simulink model "ADCSSimulator"  (R2024a)
settings: Solver=ode4  StartTime=0.0  StopTime=600  FixedStep=0.01  MaxStep=0.1  RelTol=1e-3  AbsTol=1e-3
values from neighbouring files (symbols this model uses):
  ActuatorAllocationMatrix = ActuatorPhysicalMatrix' * inv(ActuatorPhysicalMatrix * ActuatorPhysicalMatrix')    [set_Init.m]
  ActuatorPhysicalMatrix = [1, 0, 0, 0 ... (first row only)    [set_Init.m]
  albedo_irradiance = 300    [set_Init.m]
  b = 0    [set_Init.m]
  Cd = 2.2    [set_Init.m]
  h_bias = [0; 0; 0]    [set_Init.m]
  J = 4.0e-3 / 628    (= 6.36942675159e-06)    [set_Init.m]
  k_Bdot = ((4 * pi * 0.5236 * 0.0055) / (5677.2 * (4.5e-5)^2))    (= 3147.8423197)    [set_Init.m]
  K_E = K_T    (= 0.0022)    [set_Init.m]
  K_T = 0.0022    [set_Init.m]
  P0 = blkdiag(P0_att, P0_bias)    [set_Init.m]
  P0_att = eye(3) * initial_variance_rad2    [set_Init.m]
  PowerVoltageBus_01 = 3.3    [set_Init.m]
  PowerVoltageBus_02 = 3.3    [set_Init.m]
  PowerVoltageBus_03 = 3.3    [set_Init.m]
  PowerVoltageBus_04 = 3.3    [set_Init.m]
  PowerVoltageBus_05 = 3.3    [set_Init.m]
  PowerVoltageBus_06 = 3.3    [set_Init.m]
  PowerVoltageBus_07 = 3.3    [set_Init.m]
  PowerVoltageBus_08 = 3.3    [set_Init.m]
  PowerVoltageBus_09 = 3.3    [set_Init.m]
  PowerVoltageBus_10 = 3.3    [set_Init.m]
  PowerVoltageBus_11 = 3.3    [set_Init.m]
  PowerVoltageBus_12 = 0.0    (= 0)    [set_Init.m]
  PowerVoltageBus_13 = 0.0    (= 0)    [set_Init.m]
  PowerVoltageBus_14 = 0.0    (= 0)    [set_Init.m]
  PowerVoltageBus_15 = 0.0    (= 0)    [set_Init.m]
  R = 2.0    (= 2)    [set_Init.m]
  ressidual_m = [3e-4; -2e-4; 1e-4]    [set_Init.m]
  solar_irradiance = 1361    [set_Init.m]
  surface_areas = [A_xy, A_yz, A_xz, A_xy, A_yz, A_xz]    [set_Init.m]
  surface_normals_body = [eye(3) -eye(3)]    [set_Init.m]
  surface_positions_body = [       hx,   0,   0 ... (first row only)    [set_Init.m]
  surface_reflectivities = [0.9 0.8 0.9 0.9 0.9 0.9]    [set_Init.m]
  Switch_01 = 1    [set_Init.m]
  Switch_02 = 1    [set_Init.m]
  Switch_03 = 1    [set_Init.m]
  Switch_04 = 1    [set_Init.m]
  Switch_05 = 1    [set_Init.m]
  Switch_06 = 1    [set_Init.m]
  Switch_07 = 1    [set_Init.m]
  Switch_08 = 1    [set_Init.m]
  Switch_09 = 1    [set_Init.m]
  Switch_10 = 1    [set_Init.m]
  Switch_11 = 1    [set_Init.m]
  Switch_12 = 0    [set_Init.m]
  Switch_13 = 0    [set_Init.m]
  Switch_14 = 0    [set_Init.m]
  Switch_15 = 0    [set_Init.m]
  visSampleTime = 0.1    [set_Init.m]
undefined symbols (not defined in the file or in its folder): attitude, Controller, epoch, IAU, juliandate, Kd, km, Kp, m, rad, s, satellite, SGP4_parameters, simulator, UKF_parameters, WMM2020
libraries: sharedtransform x27, aerolibutil x22, aerolibconvert2 x18, simulink_extras x16, matrix_library x6, aerolibtransform2 x4, vrlib x2, aerolibgravity2 x2, aerolibobsolete x1, aerolibattitudesys x1, simulink x1
(part 5 of 8)

== system ADCSSimulator/ADCS/ADCS Hardware/Sensors/Gyroscope Model/Power Consumption Calculator ==
  note: $I_=\frac{V_{Bus}}{R} \\ P_{Consumption} =I V_{Bus}$
  Bus Voltage (V) : Inport
  Bus Creator : BusCreator  Inputs=2
  Gain1 : Gain  Gain=1/(satellite.Gyro.NominalVoltage^2/satellite.Gyro.NominalPower)
  Product : Product
  Gyro Power Consumption : Outport
  wires:
  Bus Voltage (V)/1 -> Gain1/1, Product/2
  Gain1/1 -> Product/1, Bus Creator/1  "Current (A)"
  Bus Creator/1 -> Gyro Power Consumption/1
  Product/1 -> Bus Creator/2  "Power Consumption (W)"

== system ADCSSimulator/ADCS/ADCS Hardware/Sensors/Sun Sensor Model/Init Data Wrapper ==
  Real Data : Inport
  Initial Value : Inport  Port=2
  Clock : Clock
  Switch : Switch  Threshold=1  SaturateOnIntegerOverflow=off  InputSameDT=off
  Wrapped Data : Outport
  wires:
  Clock/1 -> Switch/2
  Real Data/1 -> Switch/1
  Initial Value/1 -> Switch/3
  Switch/1 -> Wrapped Data/1

== system ADCSSimulator/ADCS/ADCS Hardware/Sensors/Sun Sensor Model/Normalizer8 ==
  A : Inport
  Divide : Product  Inputs=*/
  Dot Product : DotProduct  OutDataTypeStr=Inherit: Inherit via internal rule
  Sqrt1 : Sqrt
  Normalized(A) : Outport
  wires:
  Dot Product/1 -> Sqrt1/1
  A/1 -> Dot Product/2, Dot Product/1, Divide/1
  Sqrt1/1 -> Divide/2
  Divide/1 -> Normalized(A)/1

== system ADCSSimulator/ADCS/ADCS Hardware/Sensors/Sun Sensor Model/Power Consumption Calculator ==
  note: $I_=\frac{V_{Bus}}{R} \\ P_{Consumption} =I V_{Bus}$
  Bus Voltage (V) : Inport
  Bus Creator : BusCreator  Inputs=2
  Gain2 : Gain  Gain=1/(satellite.SS.NominalVoltage^2/satellite.SS.NominalPower)
  Product : Product
  SS Power Consumption : Outport
  wires:
  Bus Voltage (V)/1 -> Gain2/1, Product/2
  Gain2/1 -> Product/1, Bus Creator/1  "Current (A)"
  Bus Creator/1 -> SS Power Consumption/1
  Product/1 -> Bus Creator/2  "Power Consumption (W)"

== system ADCSSimulator/ADCS/ADCS Software/Attitude Control/Chart/Detumbling/Detumbling Algorithm ==
  Measured Magnetic Field [Body](T) : Inport
  Measured Angular Velocity [Body](rad/s) : Inport  Port=2
  Constant11 : Constant  Value=k_Bdot
  Cross Product : matrix_library/Cross Product
  Divide : Product  Inputs=*/
  Divide1 : Product  Inputs=*/
  Product : Product
  sqrt : Subsystem
  Detumbling: Magnetic Dipole Command : Outport
  wires:
  sqrt/1(sqrt(u)) -> Divide1/2, Divide/2  "||B||"
  Divide1/1 -> Detumbling: Magnetic Dipole Command/1  "k/||B||*omega*b"
  Product/1 -> Divide1/1  "k(omega*b)"
  Cross Product/1 -> Product/2  "omega*b"
  Divide/1 -> Cross Product/2  "b"
  Measured Angular Velocity [Body](rad/s)/1 -> Cross Product/1
  Constant11/1 -> Product/1
  Measured Magnetic Field [Body](T)/1 -> sqrt/1(u), Divide/1

== system ADCSSimulator/ADCS/ADCS Software/Attitude Control/Chart/Nadir_Pointing/Actuator Allocation & Feed-Forward ==
  m_cmd_raw_Am2 : Inport
  tau_req_Nm : Inport  Port=2
  B_meas_Body_T : Inport  Port=3
  Cross Product : matrix_library/Cross Product
  Saturation : Saturate  UpperLimit=satellite.MTQ.DPMoment  LowerLimit=-satellite.MTQ.DPMoment
  Sum : Sum  Inputs=|-+
  m_cmd_final : Outport
  tau_rw_cmd : Outport  Port=2
  wires:
  tau_req_Nm/1 -> Sum/2
  m_cmd_raw_Am2/1 -> Saturation/1
  Saturation/1 -> Cross Product/1, m_cmd_final/1
  B_meas_Body_T/1 -> Cross Product/2
  Cross Product/1 -> Sum/1
  Sum/1 -> tau_rw_cmd/1  "tau_net"

== system ADCSSimulator/ADCS/ADCS Software/Attitude Control/Chart/Nadir_Pointing/Momentum Management ==
  h_rw_Nms : Inport
  B_meas_Body_T : Inport  Port=2
  Cross Product : matrix_library/Cross Product
  Divide : Product  Inputs=*/
  Dot Product : DotProduct  OutDataTypeStr=Inherit: Inherit via internal rule
  Gain : Gain  Gain=Controller.Desat.K_desat
  Sum : Sum  Inputs=|+-
  Sum1 : Sum  Inputs=|++
  h_Desired : Constant  Value=h_bias
  h_Desired1 : Constant  Value=1e-12
  m_cmd_raw_Am2 : Outport
  wires:
  h_rw_Nms/1 -> Sum/1
  h_Desired/1 -> Sum/2
  Sum/1 -> Gain/1
  Gain/1 -> Cross Product/1  "tau_dump"
  B_meas_Body_T/1 -> Dot Product/2, Dot Product/1, Cross Product/2
  Dot Product/1 -> Sum1/1  "||B||^2"
  Sum1/1 -> Divide/2
  h_Desired1/1 -> Sum1/2
  Cross Product/1 -> Divide/1
  Divide/1 -> m_cmd_raw_Am2/1

== system ADCSSimulator/ADCS/ADCS Software/Attitude Control/Chart/Nadir_Pointing/َAttitude Controller (LQR Controller) ==
  AngularVelocity [Body] : Inport
  Body to ICRF Quaternion : Inport  Port=2
  Desired Quaternion : Inport  Port=3
  MagneticField [Body] : Inport  Port=4
  LQR Quaternion Feedback Controller : Subsystem
  PD Quaternion Feedback Controller : Subsystem  Commented=on
  q_error Calculator : Subsystem
  Nadir Pointing: Magnetic Dipole Command : Outport
  Nadir Pointing: Torque Command : Outport  Port=2
  Error Quaternion : Outport  Port=3
  wires:
  Desired Quaternion/1 -> q_error Calculator/1(q_Desired)  "q_Desired"
  LQR Quaternion Feedback Controller/1(m_Command) -> Nadir Pointing: Magnetic Dipole Command/1  "Nadir Pointing: Magnetic Dipole Command"
  LQR Quaternion Feedback Controller/2(T_Command) -> Nadir Pointing: Torque Command/1  "Nadir Pointing: Torque Command"
  q_error Calculator/1(q_Error) -> Error Quaternion/1, LQR Quaternion Feedback Controller/1(Error Quaternions [Body to Orbit])  "q_Error"
  AngularVelocity [Body]/1 -> LQR Quaternion Feedback Controller/2(AngularVelocity [Body])
  MagneticField [Body]/1 -> LQR Quaternion Feedback Controller/3(B_Body)
  Body to ICRF Quaternion/1 -> q_error Calculator/2(q_Real)  "Body to ICRF Quaternion"

== system ADCSSimulator/ADCS/ADCS Software/Attitude Control/Chart/Sun_Pointing/Sun Pointing Algorithm (LQR) ==
  Angular Velocity [Body] (T) : Inport
  Measured Magnetic Field [Body] (T) : Inport  Port=2
  ICRF to Body Quaternions : Inport  Port=3
  Desired Quaternion [Sun Pointing] : Inport  Port=4
  LQR Quaternion Feedback Controller : Subsystem
  Quaternion Inverse : aerolibutil/Quaternion Inverse
  q_error Calculator : Subsystem
  Sun Pointing: Magnetic Dipole Command : Outport
  Sun Pointing: Torque Command : Outport  Port=2
  Error Quaternion : Outport  Port=3
  wires:
  Quaternion Inverse/1 -> q_error Calculator/2(q_Real)  "Body to ICRF Quaternions"
  ICRF to Body Quaternions/1 -> Quaternion Inverse/1
  q_error Calculator/1(q_Error) -> Error Quaternion/1, LQR Quaternion Feedback Controller/1(Error Quaternions [Body to Orbit])  "q_Error"
  LQR Quaternion Feedback Controller/2(T_Command) -> Sun Pointing: Torque Command/1
  LQR Quaternion Feedback Controller/1(m_Command) -> Sun Pointing: Magnetic Dipole Command/1
  Desired Quaternion [Sun Pointing]/1 -> q_error Calculator/1(q_Desired)  "q_Desired"
  Measured Magnetic Field [Body] (T)/1 -> LQR Quaternion Feedback Controller/3(Magnetic Field [Body])
  Angular Velocity [Body] (T)/1 -> LQR Quaternion Feedback Controller/2(AngularVelocity [Body])

== system ADCSSimulator/ADCS/ADCS Software/Attitude Control/Chart/Sun_Pointing/Sun Pointing Algorithm (PD) ==
  Measured Magnetic Field [Body] (T) : Inport
  ICRF to Body Quaternions : Inport  Port=2
  Desired Quaternion [Sun Pointing] : Inport  Port=3
  PD Quaternion Feedback Controller : Subsystem
  Quaternion Inverse : aerolibutil/Quaternion Inverse
  q_error Calculator : Subsystem
  Sun Pointing: Magnetic Dipole Command : Outport
  Sun Pointing: Torque Command : Outport  Port=2
  Error Quaternion : Outport  Port=3
  wires:
  Measured Magnetic Field [Body] (T)/1 -> PD Quaternion Feedback Controller/2(Magnetic Field [Body])
  Desired Quaternion [Sun Pointing]/1 -> q_error Calculator/1(q_Desired)  "q_Desired"
  PD Quaternion Feedback Controller/1(m_command) -> Sun Pointing: Magnetic Dipole Command/1
  PD Quaternion Feedback Controller/2(T_Command) -> Sun Pointing: Torque Command/1
  q_error Calculator/1(q_Error) -> Error Quaternion/1, PD Quaternion Feedback Controller/1(q_Error)  "q_Error"
  ICRF to Body Quaternions/1 -> Quaternion Inverse/1
  Quaternion Inverse/1 -> q_error Calculator/2(q_Real)  "Body to ICRF Quaternions"

== system ADCSSimulator/ADCS/ADCS Software/Attitude Determination/Attitude Estimation Algorithm (MEKF)/Ensure Quaternion Continuity ==
  q_in : Inport
  Ensure Quaternion Continuity : MATLAB Function  TreatAsAtomicUnit=on
  Unit Delay : UnitDelay  InitialCondition=[1;0;0;0]  SampleTime=-1  HasFrameUpgradeWarning=on
  q_out : Outport
  wires:
  Ensure Quaternion Continuity/1(q_out) -> q_out/1, Unit Delay/1
  Unit Delay/1 -> Ensure Quaternion Continuity/2(q_prev)
  q_in/1 -> Ensure Quaternion Continuity/1(q_new)

== system ADCSSimulator/ADCS/ADCS Software/Attitude Determination/Attitude Estimation Algorithm (MEKF)/Ensure Quaternion Continuity1 ==
  q_in : Inport
  Ensure Quaternion Continuity : MATLAB Function  TreatAsAtomicUnit=on
  Unit Delay : UnitDelay  InitialCondition=[1;0;0;0]  SampleTime=-1  HasFrameUpgradeWarning=on
  q_out : Outport
  wires:
  Ensure Quaternion Continuity/1(q_out) -> q_out/1, Unit Delay/1
  Unit Delay/1 -> Ensure Quaternion Continuity/2(q_prev)
  q_in/1 -> Ensure Quaternion Continuity/1(q_new)

== system ADCSSimulator/ADCS/ADCS Software/Attitude Determination/Attitude Estimation Algorithm (MEKF)/Normalizer1 ==
  A : Inport
  Divide : Product  Inputs=*/
  Dot Product : DotProduct  OutDataTypeStr=Inherit: Inherit via internal rule
  Sqrt1 : Sqrt
  Normalized(A) : Outport
  wires:
  Divide/1 -> Normalized(A)/1
  Sqrt1/1 -> Divide/2
  A/1 -> Divide/1, Dot Product/1, Dot Product/2
  Dot Product/1 -> Sqrt1/1

== system ADCSSimulator/ADCS/ADCS Software/Attitude Determination/Attitude Estimation Algorithm (MEKF)/Normalizer2 ==
  A : Inport
  Divide : Product  Inputs=*/
  Dot Product : DotProduct  OutDataTypeStr=Inherit: Inherit via internal rule
  Sqrt1 : Sqrt
  Normalized(A) : Outport
  wires:
  Divide/1 -> Normalized(A)/1
  Sqrt1/1 -> Divide/2
  A/1 -> Divide/1, Dot Product/1, Dot Product/2
  Dot Product/1 -> Sqrt1/1

== system ADCSSimulator/ADCS/ADCS Software/Attitude Determination/Attitude Estimation Algorithm (MEKF)/Normalizer3 ==
  A : Inport
  Divide : Product  Inputs=*/
  Dot Product : DotProduct  OutDataTypeStr=Inherit: Inherit via internal rule
  Sqrt1 : Sqrt
  Normalized(A) : Outport
  wires:
  Dot Product/1 -> Sqrt1/1
  A/1 -> Dot Product/2, Dot Product/1, Divide/1
  Sqrt1/1 -> Divide/2
  Divide/1 -> Normalized(A)/1

== system ADCSSimulator/ADCS/ADCS Software/Attitude Determination/Attitude Estimation Algorithm (MEKF)/Normalizer8 ==
  A : Inport
  Divide : Product  Inputs=*/
  Dot Product : DotProduct  OutDataTypeStr=Inherit: Inherit via internal rule
  Sqrt1 : Sqrt
  Normalized(A) : Outport
  wires:
  Dot Product/1 -> Sqrt1/1
  A/1 -> Dot Product/2, Dot Product/1, Divide/1
  Sqrt1/1 -> Divide/2
  Divide/1 -> Normalized(A)/1

== system ADCSSimulator/ADCS/ADCS Software/Attitude Determination/Attitude Estimation Algorithm (MEKF)/Time Step Calculator ==
  Clock : Clock
  Sum : Sum  Inputs=|+-
  Unit Delay3 : UnitDelay  SampleTime=-1  HasFrameUpgradeWarning=on
  dt : Outport
  wires:
  Clock/1 -> Sum/1, Unit Delay3/1
  Unit Delay3/1 -> Sum/2
  Sum/1 -> dt/1

== system ADCSSimulator/ADCS/ADCS Software/Attitude Determination/Attitude Estimation Algorithm (MEKF)/Time Step Calculator1 ==
  Clock : Clock
  Sum : Sum  Inputs=|+-
  Unit Delay3 : UnitDelay  SampleTime=-1  HasFrameUpgradeWarning=on
  dt : Outport
  wires:
  Clock/1 -> Sum/1, Unit Delay3/1
  Unit Delay3/1 -> Sum/2
  Sum/1 -> dt/1

== system ADCSSimulator/ADCS/ADCS Software/Attitude Determination/Static Attitude Determination Algorithm (QUEST)/Ensure Quaternion Continuity1 ==
  q_in : Inport
  Ensure Quaternion Continuity : MATLAB Function  TreatAsAtomicUnit=on
  Unit Delay : UnitDelay  InitialCondition=[1;0;0;0]  SampleTime=-1  HasFrameUpgradeWarning=on
  q_out : Outport
  wires:
  Ensure Quaternion Continuity/1(q_out) -> q_out/1, Unit Delay/1
  Unit Delay/1 -> Ensure Quaternion Continuity/2(q_prev)
  q_in/1 -> Ensure Quaternion Continuity/1(q_new)

== system ADCSSimulator/ADCS/Environment Model/Reference Frames Transformations Manager/Virtual Reality World/Antenna Position to VRML ==
  x : Inport
  ECEF to VRML : Subsystem
  Length Conversion : aerolibconvert2/Length Conversion  IU=m  OU=km
  km to VRML units : Gain  Gain=1/1000
  xVRML : Outport  VectorParamsAs1DForOutWhenUnconnected=off
  wires:
  ECEF to VRML/1(VR) -> xVRML/1
  x/1 -> Length Conversion/1
  km to VRML units/1 -> ECEF to VRML/1(M)
  Length Conversion/1 -> km to VRML units/1

== system ADCSSimulator/ADCS/Environment Model/Reference Frames Transformations Manager/Virtual Reality World/Compute Antenna Properties ==
  SatScale : Inport
  Constant1 : Constant  Value=25
  Constant2 : Constant  Value=1e6
  Constant4 : Constant  Value=0
  Gain1 : Gain  Gain=.5
  Gain2 : Gain  Gain=pi/180
  Mux1 : Mux  Inputs=3
  Mux2 : Mux  Inputs=3
  Product : Product
  Selector : Selector  InputPortWidth=3  IndexOptions=Index vector (dialog)  Indices=1  OutputSizes=1
  Sum1 : Sum  Inputs=++|
  Trigonometric Function : Trigonometry  Operator=tan
  gain : Gain  Gain=.25*1e6
  AntennaScale : Outport  VectorParamsAs1DForOutWhenUnconnected=off
  AntennaTrans : Outport  Port=2  VectorParamsAs1DForOutWhenUnconnected=off
  wires:
  Selector/1 -> gain/1
  SatScale/1 -> Selector/1
  Mux1/1 -> AntennaScale/1
  Mux2/1 -> AntennaTrans/1
  Trigonometric Function/1 -> Product/1
  Gain1/1 -> Sum1/2
  Product/1 -> Mux1/1, Mux1/3
  Constant1/1 -> Gain2/1
  gain/1 -> Sum1/1
  Constant2/1 -> Product/2, Mux1/2, Gain1/1
  Sum1/1 -> Mux2/3
  Constant4/1 -> Mux2/2, Mux2/1
  Gain2/1 -> Trigonometric Function/1

== system ADCSSimulator/ADCS/Environment Model/Reference Frames Transformations Manager/Virtual Reality World/Compute Earth Rotation Rate ==
  EarthRot : Inport
  Euler Angles to Quaternions : aerolibobsolete/Euler Angles to Quaternions
  Quaternion to VRML : Subsystem
  Sum : Sum  Inputs=|++
  Unit Delay : UnitDelay  SampleTime=-1  HasFrameUpgradeWarning=on
  VRMLRot : Outport  VectorParamsAs1DForOutWhenUnconnected=off
  wires:
  Quaternion to VRML/1(AxisAngle) -> VRMLRot/1
  Euler Angles to Quaternions/1 -> Quaternion to VRML/1(q)
  Sum/1 -> Euler Angles to Quaternions/1, Unit Delay/1
  Unit Delay/1 -> Sum/2
  EarthRot/1 -> Sum/1

== system ADCSSimulator/ADCS/Environment Model/Reference Frames Transformations Manager/Virtual Reality World/Compute Umbra Translation ==
  I : Inport
  Add : Sum
  ConeHalfLength : Gain  Gain=692
  InvertSunPosECEF : Gain  Gain=-1
  unitVec : Subsystem
  O : Outport  VectorParamsAs1DForOutWhenUnconnected=off
  wires:
  unitVec/1(O) -> ConeHalfLength/1
  InvertSunPosECEF/1 -> Add/1, unitVec/1(I)
  Add/1 -> O/1
  I/1 -> InvertSunPosECEF/1
  ConeHalfLength/1 -> Add/2

== system ADCSSimulator/ADCS/Environment Model/Reference Frames Transformations Manager/Virtual Reality World/Quaternion to VRML ==
  q : Inport
  Demux : Demux
  Flip 180 deg : Constant  Commented=on  Value=[0 0 1 0]
  "Flip 180 deg, Rotate 90" : Constant  Value=[0 -.7071 .7071 0]
  Gain : Gain  Gain=2
  Mux : Mux
  Quaternion Multiplication : aerolibutil/Quaternion Multiplication
  Selector : Selector  InputPortWidth=4  IndexOptions=Index vector (dialog)  Indices=[3 4 2 1]  OutputSizes=1
  Trigonometric Function : Trigonometry  Operator=acos
  axis_angle : Outport  VectorParamsAs1DForOutWhenUnconnected=off
  wires:
  Quaternion Multiplication/1 -> Demux/1
  "Flip 180 deg, Rotate 90"/1 -> Quaternion Multiplication/2
  Demux/1 -> Trigonometric Function/1
  Trigonometric Function/1 -> Gain/1
  Mux/1 -> Selector/1
  q/1 -> Quaternion Multiplication/1
  Selector/1 -> axis_angle/1
  Gain/1 -> Mux/1
  Demux/2 -> Mux/2
  Demux/3 -> Mux/3
  Demux/4 -> Mux/4

== system ADCSSimulator/ADCS/Environment Model/Reference Frames Transformations Manager/Virtual Reality World/Quaternion to VRML1 ==
  q : Inport
  Demux : Demux
  Flip 180 deg : Constant  Value=[0 0 1 0]
  Gain : Gain  Gain=2
  Mux : Mux
  Quaternion Multiplication : aerolibutil/Quaternion Multiplication
  Selector : Selector  InputPortWidth=4  IndexOptions=Index vector (dialog)  Indices=[3 4 2 1]  OutputSizes=1
  Trigonometric Function : Trigonometry  Operator=acos
  axis_angle : Outport  VectorParamsAs1DForOutWhenUnconnected=off
  wires:
  Quaternion Multiplication/1 -> Demux/1
  q/1 -> Quaternion Multiplication/1
  Flip 180 deg/1 -> Quaternion Multiplication/2
  Demux/1 -> Trigonometric Function/1
  Trigonometric Function/1 -> Gain/1
  Mux/1 -> Selector/1
  Selector/1 -> axis_angle/1
  Gain/1 -> Mux/1
  Demux/2 -> Mux/2
  Demux/3 -> Mux/3
  Demux/4 -> Mux/4

== system ADCSSimulator/ADCS/Environment Model/Reference Frames Transformations Manager/Virtual Reality World/Radar on//off ==
  NavMode : Inport
  Add : Sum  Inputs=-+
  Compare To Constant : simulink/Logic and Bit Operations/Compare To Constant  relop===  const=1  OutDataTypeStr=boolean  ZeroCross=off
  Constant : Constant
  Data Type Conversion : DataTypeConversion  OutDataTypeStr=double  SaturateOnIntegerOverflow=off  RndMeth=Floor
  Gain : Gain  Gain=0.6
  Radar : Outport  VectorParamsAs1DForOutWhenUnconnected=off
  wires:
  Add/1 -> Radar/1
  Constant/1 -> Add/2
  Gain/1 -> Add/1
  Data Type Conversion/1 -> Gain/1
  Compare To Constant/1 -> Data Type Conversion/1
  NavMode/1 -> Compare To Constant/1

== system ADCSSimulator/ADCS/Environment Model/Reference Frames Transformations Manager/Virtual Reality World/Sat Position to VRML ==
  x : Inport
  ECEF to VRML : Subsystem
  Length Conversion : aerolibconvert2/Length Conversion  IU=m  OU=km
  km to VRML units : Gain  Gain=1/1000
  xVRML : Outport  VectorParamsAs1DForOutWhenUnconnected=off
  wires:
  Length Conversion/1 -> km to VRML units/1
  km to VRML units/1 -> ECEF to VRML/1(M)
  x/1 -> Length Conversion/1
  ECEF to VRML/1(VR) -> xVRML/1

== system ADCSSimulator/ADCS/Environment Model/Reference Frames Transformations Manager/Virtual Reality World/Satellite Model Scaling ==
  Constant : Constant  Value=2e5
  Mux : Mux  Inputs=3
  ScaleModelToVRML : Gain  Gain=1/.3e6
  Out1 : Outport  VectorParamsAs1DForOutWhenUnconnected=off
  wires:
  Mux/1 -> Out1/1
  Constant/1 -> ScaleModelToVRML/1
  ScaleModelToVRML/1 -> Mux/2, Mux/1, Mux/3

== system ADCSSimulator/ADCS/Environment Model/Reference Frames Transformations Manager/Virtual Reality World/Sun Position to VRML ==
  x : Inport
  ECEF to VRML : Subsystem
  Length Conversion : aerolibconvert2/Length Conversion  IU=m  OU=km
  km to VRML units : Gain  Gain=1/1000
  xVRML : Outport  VectorParamsAs1DForOutWhenUnconnected=off
  wires:
  Length Conversion/1 -> km to VRML units/1
  km to VRML units/1 -> ECEF to VRML/1(M)
  x/1 -> Length Conversion/1
  ECEF to VRML/1(VR) -> xVRML/1

== system ADCSSimulator/ADCS/ADCS Hardware/Actuators/Reaction Wheels Model (RWs)/Reaction Wheel Assembly/1-axis Reaction Wheel (RW#1) ==
  Command Torque [Body](N.m) : Inport
  RW Bus Voltage (V) : Inport  Port=2
  Bus Creator : BusCreator  Inputs=2
  DC Motor : Subsystem
  Flywheel : Subsystem
  Product{,1..3,5} (5 alike) : Product
  Saturation : Saturate  UpperLimit=3.2e-3  LowerLimit=-3.2e-3
  Sign3 : Signum
  Unit Delay4 : UnitDelay  SampleTime=-1  HasFrameUpgradeWarning=on
  RW Torque Out : Outport
  RW Power Consumption : Outport  Port=2
  Motor Angular Velocity (rad/s) : Outport  Port=3
  wires:
  DC Motor/1(Motor Angular Velocity (rad/s)) -> Product3/2, Flywheel/1(Motor Angular Velocity (rad/s))
  Product/1 -> Saturation/1
  Command Torque [Body](N.m)/1 -> DC Motor/1(Command Torque (N.m))
  Unit Delay4/1 -> Product5/2, Product/2, Product3/1, Product2/2
  Flywheel/1(RW Torque Out) -> Product/1
  DC Motor/2(Motor Current (A)) -> Product2/1, Product1/1  "RW Motor Current (A)"
  RW Bus Voltage (V)/1 -> Sign3/1, Product1/2
  Product1/1 -> Product5/1  "RW Motor Power Consumption (W)"
  Bus Creator/1 -> RW Power Consumption/1
  Saturation/1 -> RW Torque Out/1
  Product3/1 -> Motor Angular Velocity (rad/s)/1
  Sign3/1 -> Unit Delay4/1
  Product2/1 -> Bus Creator/1  "RW Motor Current (A)"
  Product5/1 -> Bus Creator/2  "RW Motor Power Consumption (W)"

== system ADCSSimulator/ADCS/ADCS Hardware/Actuators/Reaction Wheels Model (RWs)/Reaction Wheel Assembly/1-axis Reaction Wheel (RW#2) ==
  Command Torque [Body](N.m) : Inport
  RW Bus Voltage (V) : Inport  Port=2
  Bus Creator1 : BusCreator  Inputs=2
  DC Motor : Subsystem
  Flywheel : Subsystem
  Product{,1,3..5} (5 alike) : Product
  Saturation : Saturate  UpperLimit=3.2e-3  LowerLimit=-3.2e-3
  Sign3 : Signum
  Unit Delay4 : UnitDelay  SampleTime=-1  HasFrameUpgradeWarning=on
  RW Torque Out : Outport
  RW Power Consumption : Outport  Port=2
  Motor Angular Velocity (rad/s) : Outport  Port=3
  wires:
  DC Motor/1(Motor Angular Velocity (rad/s)) -> Product3/2, Flywheel/1(Motor Angular Velocity (rad/s))
  Product/1 -> Saturation/1
  Command Torque [Body](N.m)/1 -> DC Motor/1(Command Torque (N.m))
  Sign3/1 -> Unit Delay4/1
  Flywheel/1(RW Torque Out) -> Product/1
  DC Motor/2(Motor Current (A)) -> Product4/1, Product1/1  "RW Motor Current (A)"
  RW Bus Voltage (V)/1 -> Sign3/1, Product1/2
  Product1/1 -> Product5/1  "RW Motor Power Consumption (W)"
  Saturation/1 -> RW Torque Out/1
  Product3/1 -> Motor Angular Velocity (rad/s)/1
  Unit Delay4/1 -> Product/2, Product3/1, Product4/2, Product5/2
  Product5/1 -> Bus Creator1/2  "RW Motor Power Consumption (W)"
  Product4/1 -> Bus Creator1/1  "RW Motor Current (A)"
  Bus Creator1/1 -> RW Power Consumption/1

== system ADCSSimulator/ADCS/ADCS Hardware/Actuators/Reaction Wheels Model (RWs)/Reaction Wheel Assembly/1-axis Reaction Wheel (RW#3) ==
  Command Torque [Body](N.m) : Inport
  RW Bus Voltage (V) : Inport  Port=2
  Bus Creator1 : BusCreator  Inputs=2
  DC Motor : Subsystem
  Flywheel : Subsystem
  Product{,1,3..5} (5 alike) : Product
  Saturation : Saturate  UpperLimit=3.2e-3  LowerLimit=-3.2e-3
  Sign3 : Signum
  Unit Delay4 : UnitDelay  SampleTime=-1  HasFrameUpgradeWarning=on
  RW Torque Out : Outport
  RW Power Consumption : Outport  Port=2
  Motor Angular Velocity (rad/s) : Outport  Port=3
  wires:
  DC Motor/1(Motor Angular Velocity (rad/s)) -> Product3/2, Flywheel/1(Motor Angular Velocity (rad/s))
  Product/1 -> Saturation/1
  Command Torque [Body](N.m)/1 -> DC Motor/1(Command Torque (N.m))
  Sign3/1 -> Unit Delay4/1
  Flywheel/1(RW Torque Out) -> Product/1
  DC Motor/2(Motor Current (A)) -> Product4/1, Product1/1  "RW Motor Current (A)"
  RW Bus Voltage (V)/1 -> Sign3/1, Product1/2
  Product1/1 -> Product5/1  "RW Motor Power Consumption (W)"
  Saturation/1 -> RW Torque Out/1
  Product3/1 -> Motor Angular Velocity (rad/s)/1
  Unit Delay4/1 -> Product5/2, Product/2, Product3/1, Product4/2
  Product4/1 -> Bus Creator1/1  "RW Motor Current (A)"
  Product5/1 -> Bus Creator1/2  "RW Motor Power Consumption (W)"
  Bus Creator1/1 -> RW Power Consumption/1

== system ADCSSimulator/ADCS/ADCS Hardware/Actuators/Reaction Wheels Model (RWs)/Reaction Wheel Assembly/1-axis Reaction Wheel (RW#4) ==
  Command Torque [Body](N.m) : Inport
  RW Bus Voltage (V) : Inport  Port=2
  Bus Creator1 : BusCreator  Inputs=2
  DC Motor : Subsystem
  Flywheel : Subsystem
  Product{,1,3..5} (5 alike) : Product
  Saturation : Saturate  UpperLimit=3.2e-3  LowerLimit=-3.2e-3
  Sign3 : Signum
  Unit Delay4 : UnitDelay  SampleTime=-1  HasFrameUpgradeWarning=on
  RW Torque Out : Outport
  RW Power Consumption : Outport  Port=2
  Motor Angular Velocity (rad/s) : Outport  Port=3
  wires:
  DC Motor/1(Motor Angular Velocity (rad/s)) -> Product3/2, Flywheel/1(Motor Angular Velocity (rad/s))
  Product/1 -> Saturation/1
  Command Torque [Body](N.m)/1 -> DC Motor/1(Command Torque (N.m))
  Sign3/1 -> Unit Delay4/1
  Flywheel/1(RW Torque Out) -> Product/1
  DC Motor/2(Motor Current (A)) -> Product4/1, Product1/1  "RW Motor Current (A)"
  RW Bus Voltage (V)/1 -> Sign3/1, Product1/2
  Product1/1 -> Product5/1  "RW Motor Power Consumption (W)"
  Saturation/1 -> RW Torque Out/1
  Product3/1 -> Motor Angular Velocity (rad/s)/1
  Unit Delay4/1 -> Product5/2, Product/2, Product3/1, Product4/2
  Product4/1 -> Bus Creator1/1  "RW Motor Current (A)"
  Product5/1 -> Bus Creator1/2  "RW Motor Power Consumption (W)"
  Bus Creator1/1 -> RW Power Consumption/1

== system ADCSSimulator/ADCS/ADCS Software/Attitude Control/Chart/Detumbling/Detumbling Algorithm/sqrt ==
  u : Inport
  Dot Product : DotProduct  OutDataTypeStr=Inherit: Inherit via internal rule
  Sqrt1 : Sqrt
  sqrt(u) : Outport
  wires:
  Dot Product/1 -> Sqrt1/1
  u/1 -> Dot Product/2, Dot Product/1
  Sqrt1/1 -> sqrt(u)/1

== system ADCSSimulator/ADCS/ADCS Software/Attitude Control/Chart/Nadir_Pointing/َAttitude Controller (LQR Controller)/LQR Quaternion Feedback Controller ==
  Error Quaternions [Body to Orbit] : Inport
  AngularVelocity [Body] : Inport  Port=2
  B_Body : Inport  Port=3
  Gain : Gain  Gain=-1*Controller.LQR.K  Multiplication=Matrix(K*u)
  Mux : Mux  Inputs=2
  Product : Product
  Reshape : Reshape  OutputDimensionality=Customize  OutputDimensions=[6,1]
  Saturation : Saturate
  Selector1 : Selector  InputPortWidth=4  IndexOptions=Index vector (dialog)  Indices=[2 3 4]  OutputSizes=1
  Selector2 : Selector  InputPortWidth=4  IndexOptions=Index vector (dialog)  Indices=[1]  OutputSizes=1
  Torque to Dipole Converter : MATLAB Function  TreatAsAtomicUnit=on
  m_Command : Outport
  T_Command : Outport  Port=2
  wires:
  Gain/1 -> Saturation/1
  Mux/1 -> Reshape/1
  AngularVelocity [Body]/1 -> Mux/2
  Selector1/1 -> Product/2
  Reshape/1 -> Gain/1
  Error Quaternions [Body to Orbit]/1 -> Selector2/1, Selector1/1
  Selector2/1 -> Product/1
  Product/1 -> Mux/1
  B_Body/1 -> Torque to Dipole Converter/1(B_body)
  Saturation/1 -> Torque to Dipole Converter/2(torque_cmd_body), T_Command/1
  Torque to Dipole Converter/1(dipole_cmd_body) -> m_Command/1

== system ADCSSimulator/ADCS/ADCS Software/Attitude Control/Chart/Nadir_Pointing/َAttitude Controller (LQR Controller)/PD Quaternion Feedback Controller ==
  note: $T_{Command}=-sgn(q(0))(K_p*q_v)-K_d* \dot{q}_v$
  q_Error : Inport
  B_Body : Inport  Port=2
  Constant : Constant  Commented=on  Value=10^(-3)
  Derivative1 : Derivative
  Dipole Smoother00 : MATLAB Function  Commented=on  TreatAsAtomicUnit=on
  Kd : Gain  Gain=Kd
  Kp : Gain  Gain=Kp
  Product2 : Product
  Saturation : Saturate
  Selector : Selector  InputPortWidth=4  IndexOptions=Index vector (dialog)  Indices=[2 3 4]  OutputSizes=1
  Selector1 : Selector  InputPortWidth=4  IndexOptions=Index vector (dialog)  Indices=[1]  OutputSizes=1
  Sign1 : Signum
  Sum2 : Sum  Inputs=|++
  Terminator : Terminator  Commented=on
  Torque to Dipole Converter : MATLAB Function  TreatAsAtomicUnit=on
  m_command : Outport
  T_Command : Outport  Port=2
  wires:
  q_Error/1 -> Selector1/1, Selector/1
  B_Body/1 -> Torque to Dipole Converter/1(B_body)
  Selector/1 -> Derivative1/1, Kp/1  "q_v"
  Selector1/1 -> Sign1/1  "q(0)"
  Derivative1/1 -> Kd/1
  Sign1/1 -> Product2/1
  Kd/1 -> Sum2/2
  Product2/1 -> Sum2/1
  Sum2/1 -> Saturation/1
  Kp/1 -> Product2/2
  Torque to Dipole Converter/1(dipole_cmd_body) -> m_command/1
  Saturation/1 -> Torque to Dipole Converter/2(torque_cmd_body), T_Command/1
  Constant/1 -> Dipole Smoother00/3(k)
  Dipole Smoother00/1(m) -> Terminator/1  "M_Smooth"

== system ADCSSimulator/ADCS/ADCS Software/Attitude Control/Chart/Nadir_Pointing/َAttitude Controller (LQR Controller)/q_error Calculator ==
  note: $q_{e}=q_d ⊗ q^{-1}_{Body2ICRF}$
  q_Desired : Inport
  q_Real : Inport  Port=2
  Quaternion Conjugate : aerolibutil/Quaternion Conjugate
  Quaternion Multiplication : aerolibutil/Quaternion Multiplication
  q_Error : Outport
  wires:
  q_Desired/1 -> Quaternion Multiplication/1
  q_Real/1 -> Quaternion Conjugate/1
  Quaternion Multiplication/1 -> q_Error/1
  Quaternion Conjugate/1 -> Quaternion Multiplication/2

== system ADCSSimulator/ADCS/ADCS Software/Attitude Control/Chart/Sun_Pointing/Sun Pointing Algorithm (LQR)/LQR Quaternion Feedback Controller ==
  Error Quaternions [Body to Orbit] : Inport
  AngularVelocity [Body] : Inport  Port=2
  Magnetic Field [Body] : Inport  Port=3
  Gain : Gain  Gain=-1*Controller.LQR.K  Multiplication=Matrix(K*u)
  Mux : Mux  Inputs=2
  Product : Product
  Reshape : Reshape  OutputDimensionality=Customize  OutputDimensions=[6,1]
  Saturation : Saturate
  Selector1 : Selector  InputPortWidth=4  IndexOptions=Index vector (dialog)  Indices=[2 3 4]  OutputSizes=1
  Selector2 : Selector  InputPortWidth=4  IndexOptions=Index vector (dialog)  Indices=[1]  OutputSizes=1
  Torque to Dipole Converter : MATLAB Function  TreatAsAtomicUnit=on
  m_Command : Outport
  T_Command : Outport  Port=2
  wires:
  Gain/1 -> Saturation/1
  Mux/1 -> Reshape/1
  AngularVelocity [Body]/1 -> Mux/2
  Selector1/1 -> Product/2
  Reshape/1 -> Gain/1
  Error Quaternions [Body to Orbit]/1 -> Selector2/1, Selector1/1
  Selector2/1 -> Product/1
  Product/1 -> Mux/1
  Magnetic Field [Body]/1 -> Torque to Dipole Converter/1(B_body)
  Saturation/1 -> Torque to Dipole Converter/2(torque_cmd_body), T_Command/1
  Torque to Dipole Converter/1(dipole_cmd_body) -> m_Command/1

== system ADCSSimulator/ADCS/ADCS Software/Attitude Control/Chart/Sun_Pointing/Sun Pointing Algorithm (LQR)/q_error Calculator ==
  note: $q_{Error}=q^{-1}_{Body2ICRF}*q_{Desired}$
  q_Desired : Inport
  q_Real : Inport  Port=2
  Quaternion Inverse : aerolibutil/Quaternion Inverse
  Quaternion Multiplication : aerolibutil/Quaternion Multiplication
  q_Error : Outport
  wires:
  Quaternion Inverse/1 -> Quaternion Multiplication/2
  Quaternion Multiplication/1 -> q_Error/1
  q_Real/1 -> Quaternion Inverse/1
  q_Desired/1 -> Quaternion Multiplication/1

== system ADCSSimulator/ADCS/ADCS Software/Attitude Control/Chart/Sun_Pointing/Sun Pointing Algorithm (PD)/PD Quaternion Feedback Controller ==
  note: $T_{Command}=-sgn(q(0))(K_p*q_v)-K_d* \dot{q}_v$
  q_Error : Inport
  Magnetic Field [Body] : Inport  Port=2
  Derivative1 : Derivative
  Kd : Gain  Gain=Kd
  Kp : Gain  Gain=Kp
  Product2 : Product
  Saturation : Saturate
  Selector : Selector  InputPortWidth=4  IndexOptions=Index vector (dialog)  Indices=[2 3 4]  OutputSizes=1
  Selector1 : Selector  InputPortWidth=4  IndexOptions=Index vector (dialog)  Indices=[1]  OutputSizes=1
  Sign1 : Signum
  Sum2 : Sum  Inputs=|++
  Torque to Dipole Converter : MATLAB Function  TreatAsAtomicUnit=on
  m_command : Outport
  T_Command : Outport  Port=2
  wires:
  q_Error/1 -> Selector1/1, Selector/1
  Selector/1 -> Derivative1/1, Kp/1  "q_v"
  Selector1/1 -> Sign1/1  "q(0)"
  Derivative1/1 -> Kd/1
  Sign1/1 -> Product2/1
  Kd/1 -> Sum2/2
  Product2/1 -> Sum2/1
  Sum2/1 -> Saturation/1
  Kp/1 -> Product2/2
  Torque to Dipole Converter/1(dipole_cmd_body) -> m_command/1
  Saturation/1 -> Torque to Dipole Converter/2(torque_cmd_body), T_Command/1
  Magnetic Field [Body]/1 -> Torque to Dipole Converter/1(B_body)

== system ADCSSimulator/ADCS/ADCS Software/Attitude Control/Chart/Sun_Pointing/Sun Pointing Algorithm (PD)/q_error Calculator ==
  note: $q_{Error}=q^{-1}_{Body2ICRF}*q_{Desired}$
  q_Desired : Inport
  q_Real : Inport  Port=2
  Quaternion Inverse : aerolibutil/Quaternion Inverse
  Quaternion Multiplication : aerolibutil/Quaternion Multiplication
  q_Error : Outport
  wires:
  q_Desired/1 -> Quaternion Multiplication/1
  q_Real/1 -> Quaternion Inverse/1
  Quaternion Multiplication/1 -> q_Error/1
  Quaternion Inverse/1 -> Quaternion Multiplication/2

== system ADCSSimulator/ADCS/Environment Model/Reference Frames Transformations Manager/Virtual Reality World/Antenna Position to VRML/ECEF to VRML ==
  M : Inport  PortDimensions=3
  Selector : Selector  InputPortWidth=3  IndexOptions=Index vector (dialog)  Indices=[2 3 1]  OutputSizes=1
  VR : Outport  PortDimensions=3  VectorParamsAs1DForOutWhenUnconnected=off
  wires:
  Selector/1 -> VR/1
  M/1 -> Selector/1

== system ADCSSimulator/ADCS/Environment Model/Reference Frames Transformations Manager/Virtual Reality World/Compute Earth Rotation Rate/Quaternion to VRML ==
  q : Inport
  Demux : Demux
  Gain : Gain  Gain=2
  Gain3 : Gain  Gain=[-1 1 1 1]
  Mux : Mux
  Selector : Selector  InputPortWidth=4  IndexOptions=Index vector (dialog)  Indices=[2 4 3 1]  OutputSizes=1
  Trigonometric Function : Trigonometry  Operator=acos
  AxisAngle : Outport  VectorParamsAs1DForOutWhenUnconnected=off
  wires:
  Demux/1 -> Trigonometric Function/1
  Trigonometric Function/1 -> Gain/1
  Mux/1 -> Selector/1
  q/1 -> Demux/1
  Gain3/1 -> AxisAngle/1
  Selector/1 -> Gain3/1
  Gain/1 -> Mux/1
  Demux/2 -> Mux/2
  Demux/3 -> Mux/3
  Demux/4 -> Mux/4

== system ADCSSimulator/ADCS/Environment Model/Reference Frames Transformations Manager/Virtual Reality World/Compute Umbra Translation/unitVec ==
  I : Inport
  Divide : Product  Inputs=*/
  Dot Product : DotProduct  OutDataTypeStr=Inherit: Inherit via internal rule
  Sqrt : Sqrt
  O : Outport  VectorParamsAs1DForOutWhenUnconnected=off
  wires:
  Sqrt/1 -> Divide/2
  Divide/1 -> O/1
  I/1 -> Dot Product/2, Dot Product/1, Divide/1
  Dot Product/1 -> Sqrt/1

== system ADCSSimulator/ADCS/Environment Model/Reference Frames Transformations Manager/Virtual Reality World/Sat Position to VRML/ECEF to VRML ==
  M : Inport  PortDimensions=3
  Selector : Selector  InputPortWidth=3  IndexOptions=Index vector (dialog)  Indices=[2 3 1]  OutputSizes=1
  VR : Outport  PortDimensions=3  VectorParamsAs1DForOutWhenUnconnected=off
  wires:
  Selector/1 -> VR/1
  M/1 -> Selector/1

== system ADCSSimulator/ADCS/Environment Model/Reference Frames Transformations Manager/Virtual Reality World/Sun Position to VRML/ECEF to VRML ==
  M : Inport  PortDimensions=3
  Selector : Selector  InputPortWidth=3  IndexOptions=Index vector (dialog)  Indices=[2 3 1]  OutputSizes=1
  VR : Outport  PortDimensions=3  VectorParamsAs1DForOutWhenUnconnected=off
  wires:
  Selector/1 -> VR/1
  M/1 -> Selector/1

== system ADCSSimulator/ADCS/ADCS Hardware/Actuators/Reaction Wheels Model (RWs)/Reaction Wheel Assembly/1-axis Reaction Wheel (RW#1)/DC Motor ==
  note: $K_T: \ \text{Motor Torque Constant}\\ K_E=K_T : \ \text{Back EMF Constant}$
  Command Torque (N.m) : Inport
  Back EMF Constant : Gain  Gain=K_E
  Forward Gain : Gain  Gain=1/K_T
  Integrator : Integrator
  Integrator1 : Integrator
  Motor Torque Constant : Gain  Gain=K_T
  Reciprocal of Motor Resistance : Gain  Gain=1/R
  Reciprocal of Motor Torque Constant : Gain  Gain=1/K_T
  Reciprocal of Wheel Inertia : Gain  Gain=1/J
  Saturation : Saturate  UpperLimit=2  LowerLimit=-2
  Saturation1 : Saturate  UpperLimit=+5  LowerLimit=-5
  Saturation2 : Saturate  UpperLimit=630  LowerLimit=-630
  Scope : Scope
  Sum4 : Sum  Inputs=|+-
  Sum5 : Sum  Inputs=-+|
  Sum6 : Sum  Inputs=-+|
  Viscous Damping Coefficient : Gain  Gain=b
  Motor Angular Velocity (rad/s) : Outport
  Motor Current (A) : Outport  Port=2
  wires:
  Back EMF Constant/1 -> Scope/1, Sum5/1  "Back EMF Voltage (V)"
  Sum5/1 -> Saturation1/1  "Motor Voltage(V_M)"
  Integrator1/1 -> Forward Gain/1
  Integrator/1 -> Saturation2/1  "Motor Angular Velocity (rad/s)"
  Sum4/1 -> Integrator1/1
  Reciprocal of Motor Torque Constant/1 -> Saturation/1  "Command Current(I_C)"
  Reciprocal of Motor Resistance/1 -> Sum4/2, Motor Current (A)/1, Motor Torque Constant/1  "Motor Current(I_M)"
  Command Torque (N.m)/1 -> Reciprocal of Motor Torque Constant/1
  Forward Gain/1 -> Sum5/2  "Command Current(I_C)"
  Sum6/1 -> Reciprocal of Wheel Inertia/1  "Result Torque(T_R)"
  Motor Torque Constant/1 -> Sum6/2  "Motor Torque(M_T)"
  Reciprocal of Wheel Inertia/1 -> Integrator/1  "Motor Angular Acceleration  (rad/s^2)"
  Viscous Damping Coefficient/1 -> Sum6/1
  Saturation/1 -> Sum4/1
  Saturation1/1 -> Reciprocal of Motor Resistance/1
  Saturation2/1 -> Motor Angular Velocity (rad/s)/1, Back EMF Constant/1, Viscous Damping Coefficient/1

== system ADCSSimulator/ADCS/ADCS Hardware/Actuators/Reaction Wheels Model (RWs)/Reaction Wheel Assembly/1-axis Reaction Wheel (RW#1)/Flywheel ==
  Motor Angular Velocity (rad/s) : Inport
  Derivative : Derivative
  Wheel Inertia : Gain  Gain=J
  RW Torque Out : Outport
  wires:
  Motor Angular Velocity (rad/s)/1 -> Derivative/1
  Derivative/1 -> Wheel Inertia/1  "Motor Angular Acceleration (rad/s^2)"
  Wheel Inertia/1 -> RW Torque Out/1

== system ADCSSimulator/ADCS/ADCS Hardware/Actuators/Reaction Wheels Model (RWs)/Reaction Wheel Assembly/1-axis Reaction Wheel (RW#2)/DC Motor ==
  note: $K_T: \ \text{Motor Torque Constant}\\ K_E=K_T : \ \text{Back EMF Constant}$
  Command Torque (N.m) : Inport
  Back EMF Constant : Gain  Gain=K_E
  Forward Gain : Gain  Gain=1/K_T
  Integrator : Integrator
  Integrator1 : Integrator
  Motor Torque Constant : Gain  Gain=K_T
  Reciprocal of Motor Resistance : Gain  Gain=1/R
  Reciprocal of Motor Torque Constant : Gain  Gain=1/K_T
  Reciprocal of Wheel Inertia : Gain  Gain=1/J
  Saturation : Saturate  UpperLimit=2  LowerLimit=-2
  Saturation1 : Saturate  UpperLimit=+5  LowerLimit=-5
  Saturation2 : Saturate  UpperLimit=630  LowerLimit=-630
  Scope : Scope
  Sum4 : Sum  Inputs=|+-
  Sum5 : Sum  Inputs=-+|
  Sum6 : Sum  Inputs=-+|
  Viscous Damping Coefficient : Gain  Gain=b
  Motor Angular Velocity (rad/s) : Outport
  Motor Current (A) : Outport  Port=2
  wires:
  Back EMF Constant/1 -> Scope/1, Sum5/1  "Back EMF Voltage (V)"
  Sum5/1 -> Saturation1/1  "Motor Voltage(V_M)"
  Integrator1/1 -> Forward Gain/1
  Integrator/1 -> Saturation2/1  "Motor Angular Velocity (rad/s)"
  Sum4/1 -> Integrator1/1
  Reciprocal of Motor Torque Constant/1 -> Saturation/1  "Command Current(I_C)"
  Reciprocal of Motor Resistance/1 -> Sum4/2, Motor Current (A)/1, Motor Torque Constant/1  "Motor Current(I_M)"
  Command Torque (N.m)/1 -> Reciprocal of Motor Torque Constant/1
  Forward Gain/1 -> Sum5/2  "Command Current(I_C)"
  Sum6/1 -> Reciprocal of Wheel Inertia/1  "Result Torque(T_R)"
  Motor Torque Constant/1 -> Sum6/2  "Motor Torque(M_T)"
  Reciprocal of Wheel Inertia/1 -> Integrator/1  "Motor Angular Acceleration  (rad/s^2)"
  Viscous Damping Coefficient/1 -> Sum6/1
  Saturation/1 -> Sum4/1
  Saturation1/1 -> Reciprocal of Motor Resistance/1
  Saturation2/1 -> Motor Angular Velocity (rad/s)/1, Back EMF Constant/1, Viscous Damping Coefficient/1

== system ADCSSimulator/ADCS/ADCS Hardware/Actuators/Reaction Wheels Model (RWs)/Reaction Wheel Assembly/1-axis Reaction Wheel (RW#2)/Flywheel ==
  Motor Angular Velocity (rad/s) : Inport
  Derivative : Derivative
  Wheel Inertia : Gain  Gain=J
  RW Torque Out : Outport
  wires:
  Motor Angular Velocity (rad/s)/1 -> Derivative/1
  Derivative/1 -> Wheel Inertia/1  "Motor Angular Acceleration (rad/s^2)"
  Wheel Inertia/1 -> RW Torque Out/1

== system ADCSSimulator/ADCS/ADCS Hardware/Actuators/Reaction Wheels Model (RWs)/Reaction Wheel Assembly/1-axis Reaction Wheel (RW#3)/DC Motor ==
  note: $K_T: \ \text{Motor Torque Constant}\\ K_E=K_T : \ \text{Back EMF Constant}$
  Command Torque (N.m) : Inport
  Back EMF Constant : Gain  Gain=K_E
  Forward Gain : Gain  Gain=1/K_T
  Integrator : Integrator
  Integrator1 : Integrator
  Motor Torque Constant : Gain  Gain=K_T
  Reciprocal of Motor Resistance : Gain  Gain=1/R
  Reciprocal of Motor Torque Constant : Gain  Gain=1/K_T
  Reciprocal of Wheel Inertia : Gain  Gain=1/J
  Saturation : Saturate  UpperLimit=2  LowerLimit=-2
  Saturation1 : Saturate  UpperLimit=+5  LowerLimit=-5
  Saturation2 : Saturate  UpperLimit=630  LowerLimit=-630
  Scope : Scope
  Sum4 : Sum  Inputs=|+-
  Sum5 : Sum  Inputs=-+|
  Sum6 : Sum  Inputs=-+|
  Viscous Damping Coefficient : Gain  Gain=b
  Motor Angular Velocity (rad/s) : Outport
  Motor Current (A) : Outport  Port=2
  wires:
  Back EMF Constant/1 -> Scope/1, Sum5/1  "Back EMF Voltage (V)"
  Sum5/1 -> Saturation1/1  "Motor Voltage(V_M)"
  Integrator1/1 -> Forward Gain/1
  Integrator/1 -> Saturation2/1  "Motor Angular Velocity (rad/s)"
  Sum4/1 -> Integrator1/1
  Reciprocal of Motor Torque Constant/1 -> Saturation/1  "Command Current(I_C)"
  Reciprocal of Motor Resistance/1 -> Sum4/2, Motor Current (A)/1, Motor Torque Constant/1  "Motor Current(I_M)"
  Command Torque (N.m)/1 -> Reciprocal of Motor Torque Constant/1
  Forward Gain/1 -> Sum5/2  "Command Current(I_C)"
  Sum6/1 -> Reciprocal of Wheel Inertia/1  "Result Torque(T_R)"
  Motor Torque Constant/1 -> Sum6/2  "Motor Torque(M_T)"
  Reciprocal of Wheel Inertia/1 -> Integrator/1  "Motor Angular Acceleration  (rad/s^2)"
  Viscous Damping Coefficient/1 -> Sum6/1
  Saturation/1 -> Sum4/1
  Saturation1/1 -> Reciprocal of Motor Resistance/1
  Saturation2/1 -> Motor Angular Velocity (rad/s)/1, Back EMF Constant/1, Viscous Damping Coefficient/1

== system ADCSSimulator/ADCS/ADCS Hardware/Actuators/Reaction Wheels Model (RWs)/Reaction Wheel Assembly/1-axis Reaction Wheel (RW#3)/Flywheel ==
  Motor Angular Velocity (rad/s) : Inport
  Derivative : Derivative
  Wheel Inertia : Gain  Gain=J
  RW Torque Out : Outport
  wires:
  Motor Angular Velocity (rad/s)/1 -> Derivative/1
  Derivative/1 -> Wheel Inertia/1  "Motor Angular Acceleration (rad/s^2)"
  Wheel Inertia/1 -> RW Torque Out/1

== system ADCSSimulator/ADCS/ADCS Hardware/Actuators/Reaction Wheels Model (RWs)/Reaction Wheel Assembly/1-axis Reaction Wheel (RW#4)/DC Motor ==
  note: $K_T: \ \text{Motor Torque Constant}\\ K_E=K_T : \ \text{Back EMF Constant}$
  Command Torque (N.m) : Inport
  Back EMF Constant : Gain  Gain=K_E
  Forward Gain : Gain  Gain=1/K_T
  Integrator : Integrator
  Integrator1 : Integrator
  Motor Torque Constant : Gain  Gain=K_T
  Reciprocal of Motor Resistance : Gain  Gain=1/R
  Reciprocal of Motor Torque Constant : Gain  Gain=1/K_T
  Reciprocal of Wheel Inertia : Gain  Gain=1/J
  Saturation : Saturate  UpperLimit=2  LowerLimit=-2
  Saturation1 : Saturate  UpperLimit=+5  LowerLimit=-5
  Saturation2 : Saturate  UpperLimit=630  LowerLimit=-630
  Scope : Scope
  Sum4 : Sum  Inputs=|+-
  Sum5 : Sum  Inputs=-+|
  Sum6 : Sum  Inputs=-+|
  Viscous Damping Coefficient : Gain  Gain=b
  Motor Angular Velocity (rad/s) : Outport
  Motor Current (A) : Outport  Port=2
  wires:
  Back EMF Constant/1 -> Scope/1, Sum5/1  "Back EMF Voltage (V)"
  Sum5/1 -> Saturation1/1  "Motor Voltage(V_M)"
  Integrator1/1 -> Forward Gain/1
  Integrator/1 -> Saturation2/1  "Motor Angular Velocity (rad/s)"
  Sum4/1 -> Integrator1/1
  Reciprocal of Motor Torque Constant/1 -> Saturation/1  "Command Current(I_C)"
  Reciprocal of Motor Resistance/1 -> Sum4/2, Motor Current (A)/1, Motor Torque Constant/1  "Motor Current(I_M)"
  Command Torque (N.m)/1 -> Reciprocal of Motor Torque Constant/1
  Forward Gain/1 -> Sum5/2  "Command Current(I_C)"
  Sum6/1 -> Reciprocal of Wheel Inertia/1  "Result Torque(T_R)"
  Motor Torque Constant/1 -> Sum6/2  "Motor Torque(M_T)"
  Reciprocal of Wheel Inertia/1 -> Integrator/1  "Motor Angular Acceleration  (rad/s^2)"
  Viscous Damping Coefficient/1 -> Sum6/1
  Saturation/1 -> Sum4/1
  Saturation1/1 -> Reciprocal of Motor Resistance/1
  Saturation2/1 -> Motor Angular Velocity (rad/s)/1, Back EMF Constant/1, Viscous Damping Coefficient/1

== system ADCSSimulator/ADCS/ADCS Hardware/Actuators/Reaction Wheels Model (RWs)/Reaction Wheel Assembly/1-axis Reaction Wheel (RW#4)/Flywheel ==
  Motor Angular Velocity (rad/s) : Inport
  Derivative : Derivative
  Wheel Inertia : Gain  Gain=J
  RW Torque Out : Outport
  wires:
  Motor Angular Velocity (rad/s)/1 -> Derivative/1
  Derivative/1 -> Wheel Inertia/1  "Motor Angular Acceleration (rad/s^2)"
  Wheel Inertia/1 -> RW Torque Out/1

== matlab function ADCSSimulator/ADCS/Environment Model/Disturbance Calculator/Gravity Gradient/MATLAB Function ==
  data: Rearth_body input; gravity_gradient_torque output; J input
function gravity_gradient_torque = gravity_Gradient_Torque(Rearth_body, J)
% GRAVITY_GRADIENT_TORQUE calculates the gravity gradient torque on a satellite
% in the body frame using the simplified cross-product formula.
%
% Inputs:
%   Rearth_body : [3x1] Satellite position vector in body frame [m]
%   J           : [3x3] Satellite inertia tensor in body frame [kg·m^2]
%
% Output:
%   gravity_gradient_torque : [3x1] Gravity gradient torque in body frame [N·m]

% Earth's gravitational parameter [m^3/s^2]
mu = 3.986004418e14;

% Magnitude of position vector
r = norm(Rearth_body);

% Unit vector along the position vector
r_hat = Rearth_body / r;

% Gravity gradient torque (in body frame)
gravity_gradient_torque = (3 * mu / r^3) * cross(r_hat, J * r_hat);

end

== matlab function ADCSSimulator/ADCS/Environment Model/Disturbance Calculator/Solar Radiation Pressure (SRP)/MATLAB Function ==
  data: sun_vector_body input; SRP_Torque output; surface_normals_body input; surface_areas input; surface_reflectivities input; surface_positions_body input; solar_irradiance input
function SRP_Torque = SRP(sun_vector_body, ...
    surface_normals_body, ...
    surface_areas, ...
    surface_reflectivities, ...
    surface_positions_body, ...
    solar_irradiance)
% SRP Calculates the Solar Radiation Pressure (SRP) torque on a satellite
%
% Inputs:
%   sun_vector_body         : [3x1] Sun direction in body frame (unit vector)
%   surface_normals_body    : [3x6] Surface normal vectors in body frame
%   surface_areas           : [1x6] Surface areas [m^2]
%   surface_reflectivities  : [1x6] Surface reflectivity coefficients [0–1]
%   surface_positions_body  : [3x6] Position vectors from CoM to surface centers [m]
%   solar_irradiance        : [scalar] Solar irradiance [W/m^2]
%
% Output:
%   SRP_Torque              : [3x1] Resultant SRP torque in body frame [Nm]

% Constants
c = 299792458;                  % Speed of light [m/s]
P = solar_irradiance / c;       % Solar radiation pressure [Pa]

% Normalize sun vector
sun_unit = sun_vector_body / norm(sun_vector_body);

% Initialize force matrix
F_srp = zeros(3, 6);

for i = 1:6
    n_i = surface_normals_body(:, i);
    r_i = surface_positions_body(:, i);
    A_i = surface_areas(i);
    R_i = surface_reflectivities(i);
    
    dot_proj = dot(n_i, sun_unit);
    
    if dot_proj > 0
        % Pressure force magnitude
        F_mag = -P * A_i * dot_proj;

        % SRP force direction: absorbed and reflected parts
        F_dir = (1 - R_i) * sun_unit + ...
                R_i * (2 * dot_proj * n_i + (2/3) * n_i);
        
        % Force on surface
        F_srp(:, i) = F_mag * F_dir;
    end
end

% Compute torques and sum
torques = cross(surface_positions_body, F_srp);
SRP_Torque = sum(torques, 2);

end
